simulink model "Modelo_Omnirover"  (R2026b)
settings: Solver=ode23t  StopTime=100
InitFcn:
  | %% Modelo Proyecto Omnriover - Hermes
  | clc;
  | clear;
  | 
  | % Variables de Sim
  | step_time = 1;
  | % initial_val = 10;
  | 
  | % Max Val = 7-8 rad/s
  | 
  | w1_val = 7.2; % M1 delantero izquierdo
  | w2_val = 7.2; % M2 delantero derecho
  | w3_val = 7.2; % M3 trasero izquierdo
  | w4_val = 7.2; % M4 trasero derecho
  | final_val = 0;
  | sample_time = 100;
  | 
  | % Condiciones Iniciales
  | x0 = [0; 0; 0];
  | 
  | 
  | %% PID
  | % Simulacion de Motor
  | V_nom = 12; % V
  | Vel_nom_150rpm = 100; % RPM
  | Vel_nom_140rpm = 70; % RPM
  | 
  | W_nom_150rpm = Vel_nom_150rpm * (2*pi) * (1/60);
  | W_nom_140rpm = Vel_nom_140rpm * (2*pi) * (1/60);
  | K_150 = W_nom_150rpm/V_nom;
  | K_140 = W_nom_140rpm/V_nom;
  | 
  | tao = 0.1; % entre 50 - 200 ms
  | 
  | % Ganancias PIDs
  | N = 100;
  | Kp1 = 0; % Robustez 1.5
  | Ki1 = 4.35; % 200 works
  | Kd1 = 0.005;
  | 
  | Kp2 = 0;
  | Ki2 = 3;
  | Kd2 = 0.005;
  | 
  | Kp3 = 0;
  | Ki3 = 3;
  | Kd3 = 0.005;
  | 
  | Kp4 = 0;
  | Ki4 = 3;
  | Kd4 = 0.005;
libraries: slpidlib x4
settings Model: Creator=dbarraga  LastModifiedBy=dbarraga

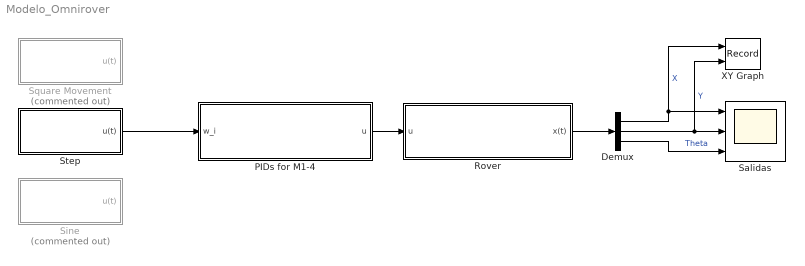
== system Modelo_Omnirover ==
  Demux : Demux  Outputs=3
  PIDs for M1-4 : Subsystem
  Rover : Subsystem
  Salidas : Scope  NumInputPorts=3
      settings: ActiveDisplayYMinimum=-3.586291147206452  ActiveDisplayYMaximum=32.276620324858079
  Sine : Subsystem  Commented=on
  Square Movement : Subsystem  Commented=on
  Step : Subsystem
  XY Graph : Record  NumPorts=2.0  FileSettingsInternal="{\"entries\":[{\"content\":{\"excelSettings\":{\"content\":{},\"type\":\"Streamout.ExcelSettings\"},\"parquetSettings\":{\"content\":{},\"type\":\"Streamout.ParquetSettings\"}},\"type\":\"Streamout.FileSettingStorage\",\"uuid\":\"\"}],\"packageUris\":[\"http:\\/\\/schema.mathworks.com\\/mf0\\/streamout_blocks\\/R2020a\"],\"version\":\"1.0\"}"  FrameSettings=[0, 0]  Layout=[1 1]  SignalsInternal="{\"entries\":[{\"content\":{\"signals\":[{\"content\":{\"blockPath\":[],\"dimensions\":[1,1],\"domain\":\"\",\"lineColor\":\"#a2142f\",\"plots\":[ 1 ],\"port\":1,\"sid\":[\"\"],\"signalID\":1,\"signalName\":\"X\"},\"type\":\"RecordBlkView.Signal\",\"uuid\":\"\"},{\"content\":{\"blockPath\":[],\"dimensions\":[1,1],\"domain\":\"\",\"lineColor\":\"#139fff\",\"plots\":[ 1 ],\"port\":2,\"sid\":[\"\"],\"signalID\":2,\"signalName\":\"Y\"},\"type\":\"RecordBlkView.Signal\",\"uuid\":\"\"}]},\"type\":\"RecordBlkView.InputSignals\",\"uuid\":\"\"}],\"packageUris\":[\"http:\\/\\/schema.mathworks.com\\/mf0\\/streamout_blocks\\/R2020a\"],\"version\":\"1.0\"}"  VisualizationBindings="{\"xyplotplugin\":{\"info\":[{\"series\":[{\"bindingParametersList\":[{\"parameter\":\"X-Axis\",\"signalID\":2,\"signalName\":\"Y\"},{\"parameter\":\"Y-Axis\",\"signalID\":1,\"signalName\":\"X\"}],\"seriesID\":0}],\"subplotID\":1}]}}"  CompatibilityTag=XY
  wires:
  Demux/2 -> XY Graph/2, Salidas/2  "Y"
  Demux/1 -> XY Graph/1, Salidas/1  "X"
  Demux/3 -> Salidas/3  "Theta"
  Rover/1(x(t)) -> Demux/1
  PIDs for M1-4/1(u) -> Rover/1(u)
  Step/1(u(t)) -> PIDs for M1-4/1(w_i)

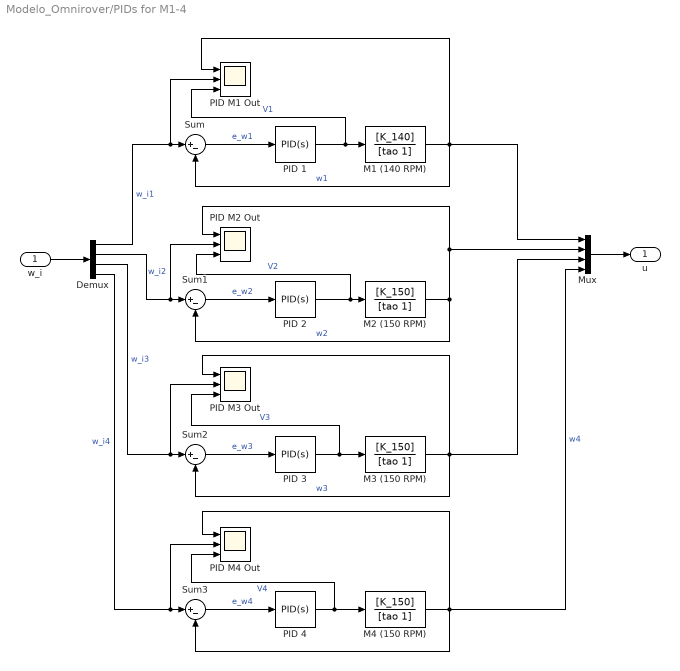
== system Modelo_Omnirover/PIDs for M1-4 ==
  w_i : Inport
  Demux : Demux
  M1 (140 RPM) : TransferFcn  Numerator=[K_140]  Denominator=[tao 1]
  M2 (150 RPM) : TransferFcn  Numerator=[K_150]  Denominator=[tao 1]
  M3 (150 RPM) : TransferFcn  Numerator=[K_150]  Denominator=[tao 1]
  M4 (150 RPM) : TransferFcn  Numerator=[K_150]  Denominator=[tao 1]
  Mux : Mux
  PID 1 : slpidlib/PID Controller  Controller=PID  Form=Parallel  TimeDomain=Continuous-time  UseExternalTs=off  SampleTime=-1  IntegratorMethod=Forward Euler  FilterMethod=Forward Euler  ControllerParametersSource=internal  P=Kp1  I=Ki1  UseKiTs=off  D=Kd1  UseExternalDerivativeSource=off  N=N  UseFilter=on  TunerSelectOption=Transfer Function Based (PID Tuner App)  InitialConditionSource=internal  InitialConditionForIntegrator=0  InitialConditionForFilter=0  DifferentiatorICPrevScaledInput=0  ExternalReset=none  TrackingMode=off  Kt=1  LimitOutput=off  SatLimitsSource=internal  UpperSaturationLimit=inf  LowerSaturationLimit=-inf  LinearizeAsGain=on  AntiWindupMode=none  Kb=1  LimitIntegrator=off  UpperIntegratorSaturationLimit=inf  LowerIntegratorSaturationLimit=-inf  POutMin=[]  POutMax=[]  IOutMin=[]  IOutMax=[]  DOutMin=[]  DOutMax=[]  NOutMin=[]  NOutMax=[]  SumOutMin=[]  SumOutMax=[]  SaturationOutMin=[]  SaturationOutMax=[]  PParamMin=[]  PParamMax=[]  IParamMin=[]  IParamMax=[]  DParamMin=[]  DParamMax=[]  NParamMin=[]  NParamMax=[]  KbParamMin=[]  KbParamMax=[]  KtParamMin=[]  KtParamMax=[]  KbOutMin=[]  KbOutMax=[]  KtOutMin=[]  KtOutMax=[]  IntegratorOutMin=[]  IntegratorOutMax=[]  FilterOutMin=[]  FilterOutMax=[]  SumI1OutMin=[]  SumI1OutMax=[]  SumI2OutMin=[]  SumI2OutMax=[]  SumI3OutMin=[]  SumI3OutMax=[]  SumI4OutMin=[]  SumI4OutMax=[]  SumDOutMin=[]  SumDOutMax=[]  DifferentiatorOutMin=[]  DifferentiatorOutMax=[]  FilterDiffOutCoefMin=[]  FilterDiffOutCoefMax=[]  ReciprocalOutMin=[]  ReciprocalOutMax=[]  SumDenOutMin=[]  SumDenOutMax=[]  SumNumOutMin=[]  SumNumOutMax=[]  DivideOutMin=[]  DivideOutMax=[]  UdiffTsProdOutMin=[]  UdiffTsProdOutMax=[]  NTsProdOutMin=[]  NTsProdOutMax=[]  UintegralTsProdOutMin=[]  UintegralTsProdOutMax=[]  UngainTsProdOutMin=[]  UngainTsProdOutMax=[]  ClampingZeroOutDataTypeStr=Inherit: Inherit via back propagation  ClampingZeroOutMin=[]  ClampingZeroOutMax=[]  FilterDenConstantOutDataTypeStr=Inherit: Inherit via back propagation  FilterDenConstantOutMin=[]  FilterDenConstantOutMax=[]  PCopyOutDataTypeStr=Inherit: Inherit via back propagation  PCopyOutMin=[]  PCopyOutMax=[]  NCopyOutDataTypeStr=Inherit: Inherit via back propagation  NCopyOutMin=[]  NCopyOutMax=[]  IntegratorContinuousStateAttributes=''  IntegratorStateMustResolveToSignalObject=off  IntegratorRTWStateStorageClass=Auto  FilterContinuousStateAttributes=''  FilterStateMustResolveToSignalObject=off  FilterRTWStateStorageClass=Auto  ParallelPVariant=InternalParameters  IdealPVariant=Disabled  IVariant=InternalParameters  DVariant=InternalParameters  IntegratorVariant=Continuous  SatVariant=Disabled  AWVariant=Passthrough  PCopyVariant=Disabled  TRVariant=Disabled  FdbkBlocksVariant=Forward  IdealPFdbkVariant=Disabled  SatFdbkVariant=Disabled  DerivativeFilterVariant=ContFilter  NVariant=InternalParameters  NCopyVariant=Disabled  FilterICVariant=InternalICsFilter  IntegratorICVariant=InternalICs  ExternalResetVariant=Disabled  TRSumVariant=Passthrough  SumFdbkVariant=Disabled  SumVariant=Sum_PID  TsampFilterVariant=InternalTs  TsampNgainVariant=Passthrough  TsampIntegralVariant=Disabled_SignalSpec  ExternalSaturationOutDataTypeStr=Inherit: Same as second input  DerivativeSourceVariant=ErrorSignal  PreIntVariant=InternalPreInt
  PID 2 : slpidlib/PID Controller  Controller=PID  Form=Parallel  TimeDomain=Continuous-time  UseExternalTs=off  SampleTime=-1  IntegratorMethod=Forward Euler  FilterMethod=Forward Euler  ControllerParametersSource=internal  P=Kp2  I=Ki2  UseKiTs=off  D=Kd2  UseExternalDerivativeSource=off  N=N  UseFilter=on  TunerSelectOption=Transfer Function Based (PID Tuner App)  InitialConditionSource=internal  InitialConditionForIntegrator=0  InitialConditionForFilter=0  DifferentiatorICPrevScaledInput=0  ExternalReset=none  TrackingMode=off  Kt=1  LimitOutput=off  SatLimitsSource=internal  UpperSaturationLimit=inf  LowerSaturationLimit=-inf  LinearizeAsGain=on  AntiWindupMode=none  Kb=1  LimitIntegrator=off  UpperIntegratorSaturationLimit=inf  LowerIntegratorSaturationLimit=-inf  POutMin=[]  POutMax=[]  IOutMin=[]  IOutMax=[]  DOutMin=[]  DOutMax=[]  NOutMin=[]  NOutMax=[]  SumOutMin=[]  SumOutMax=[]  SaturationOutMin=[]  SaturationOutMax=[]  PParamMin=[]  PParamMax=[]  IParamMin=[]  IParamMax=[]  DParamMin=[]  DParamMax=[]  NParamMin=[]  NParamMax=[]  KbParamMin=[]  KbParamMax=[]  KtParamMin=[]  KtParamMax=[]  KbOutMin=[]  KbOutMax=[]  KtOutMin=[]  KtOutMax=[]  IntegratorOutMin=[]  IntegratorOutMax=[]  FilterOutMin=[]  FilterOutMax=[]  SumI1OutMin=[]  SumI1OutMax=[]  SumI2OutMin=[]  SumI2OutMax=[]  SumI3OutMin=[]  SumI3OutMax=[]  SumI4OutMin=[]  SumI4OutMax=[]  SumDOutMin=[]  SumDOutMax=[]  DifferentiatorOutMin=[]  DifferentiatorOutMax=[]  FilterDiffOutCoefMin=[]  FilterDiffOutCoefMax=[]  ReciprocalOutMin=[]  ReciprocalOutMax=[]  SumDenOutMin=[]  SumDenOutMax=[]  SumNumOutMin=[]  SumNumOutMax=[]  DivideOutMin=[]  DivideOutMax=[]  UdiffTsProdOutMin=[]  UdiffTsProdOutMax=[]  NTsProdOutMin=[]  NTsProdOutMax=[]  UintegralTsProdOutMin=[]  UintegralTsProdOutMax=[]  UngainTsProdOutMin=[]  UngainTsProdOutMax=[]  ClampingZeroOutDataTypeStr=Inherit: Inherit via back propagation  ClampingZeroOutMin=[]  ClampingZeroOutMax=[]  FilterDenConstantOutDataTypeStr=Inherit: Inherit via back propagation  FilterDenConstantOutMin=[]  FilterDenConstantOutMax=[]  PCopyOutDataTypeStr=Inherit: Inherit via back propagation  PCopyOutMin=[]  PCopyOutMax=[]  NCopyOutDataTypeStr=Inherit: Inherit via back propagation  NCopyOutMin=[]  NCopyOutMax=[]  IntegratorContinuousStateAttributes=''  IntegratorStateMustResolveToSignalObject=off  IntegratorRTWStateStorageClass=Auto  FilterContinuousStateAttributes=''  FilterStateMustResolveToSignalObject=off  FilterRTWStateStorageClass=Auto  ParallelPVariant=InternalParameters  IdealPVariant=Disabled  IVariant=InternalParameters  DVariant=InternalParameters  IntegratorVariant=Continuous  SatVariant=Disabled  AWVariant=Passthrough  PCopyVariant=Disabled  TRVariant=Disabled  FdbkBlocksVariant=Forward  IdealPFdbkVariant=Disabled  SatFdbkVariant=Disabled  DerivativeFilterVariant=ContFilter  NVariant=InternalParameters  NCopyVariant=Disabled  FilterICVariant=InternalICsFilter  IntegratorICVariant=InternalICs  ExternalResetVariant=Disabled  TRSumVariant=Passthrough  SumFdbkVariant=Disabled  SumVariant=Sum_PID  TsampFilterVariant=InternalTs  TsampNgainVariant=Passthrough  TsampIntegralVariant=Disabled_SignalSpec  ExternalSaturationOutDataTypeStr=Inherit: Same as second input  DerivativeSourceVariant=ErrorSignal  PreIntVariant=InternalPreInt
  PID 3 : slpidlib/PID Controller  Controller=PID  Form=Parallel  TimeDomain=Continuous-time  UseExternalTs=off  SampleTime=-1  IntegratorMethod=Forward Euler  FilterMethod=Forward Euler  ControllerParametersSource=internal  P=Kp3  I=Ki3  UseKiTs=off  D=Kd3  UseExternalDerivativeSource=off  N=N  UseFilter=on  TunerSelectOption=Transfer Function Based (PID Tuner App)  InitialConditionSource=internal  InitialConditionForIntegrator=0  InitialConditionForFilter=0  DifferentiatorICPrevScaledInput=0  ExternalReset=none  TrackingMode=off  Kt=1  LimitOutput=off  SatLimitsSource=internal  UpperSaturationLimit=inf  LowerSaturationLimit=-inf  LinearizeAsGain=on  AntiWindupMode=none  Kb=1  LimitIntegrator=off  UpperIntegratorSaturationLimit=inf  LowerIntegratorSaturationLimit=-inf  POutMin=[]  POutMax=[]  IOutMin=[]  IOutMax=[]  DOutMin=[]  DOutMax=[]  NOutMin=[]  NOutMax=[]  SumOutMin=[]  SumOutMax=[]  SaturationOutMin=[]  SaturationOutMax=[]  PParamMin=[]  PParamMax=[]  IParamMin=[]  IParamMax=[]  DParamMin=[]  DParamMax=[]  NParamMin=[]  NParamMax=[]  KbParamMin=[]  KbParamMax=[]  KtParamMin=[]  KtParamMax=[]  KbOutMin=[]  KbOutMax=[]  KtOutMin=[]  KtOutMax=[]  IntegratorOutMin=[]  IntegratorOutMax=[]  FilterOutMin=[]  FilterOutMax=[]  SumI1OutMin=[]  SumI1OutMax=[]  SumI2OutMin=[]  SumI2OutMax=[]  SumI3OutMin=[]  SumI3OutMax=[]  SumI4OutMin=[]  SumI4OutMax=[]  SumDOutMin=[]  SumDOutMax=[]  DifferentiatorOutMin=[]  DifferentiatorOutMax=[]  FilterDiffOutCoefMin=[]  FilterDiffOutCoefMax=[]  ReciprocalOutMin=[]  ReciprocalOutMax=[]  SumDenOutMin=[]  SumDenOutMax=[]  SumNumOutMin=[]  SumNumOutMax=[]  DivideOutMin=[]  DivideOutMax=[]  UdiffTsProdOutMin=[]  UdiffTsProdOutMax=[]  NTsProdOutMin=[]  NTsProdOutMax=[]  UintegralTsProdOutMin=[]  UintegralTsProdOutMax=[]  UngainTsProdOutMin=[]  UngainTsProdOutMax=[]  ClampingZeroOutDataTypeStr=Inherit: Inherit via back propagation  ClampingZeroOutMin=[]  ClampingZeroOutMax=[]  FilterDenConstantOutDataTypeStr=Inherit: Inherit via back propagation  FilterDenConstantOutMin=[]  FilterDenConstantOutMax=[]  PCopyOutDataTypeStr=Inherit: Inherit via back propagation  PCopyOutMin=[]  PCopyOutMax=[]  NCopyOutDataTypeStr=Inherit: Inherit via back propagation  NCopyOutMin=[]  NCopyOutMax=[]  IntegratorContinuousStateAttributes=''  IntegratorStateMustResolveToSignalObject=off  IntegratorRTWStateStorageClass=Auto  FilterContinuousStateAttributes=''  FilterStateMustResolveToSignalObject=off  FilterRTWStateStorageClass=Auto  ParallelPVariant=InternalParameters  IdealPVariant=Disabled  IVariant=InternalParameters  DVariant=InternalParameters  IntegratorVariant=Continuous  SatVariant=Disabled  AWVariant=Passthrough  PCopyVariant=Disabled  TRVariant=Disabled  FdbkBlocksVariant=Forward  IdealPFdbkVariant=Disabled  SatFdbkVariant=Disabled  DerivativeFilterVariant=ContFilter  NVariant=InternalParameters  NCopyVariant=Disabled  FilterICVariant=InternalICsFilter  IntegratorICVariant=InternalICs  ExternalResetVariant=Disabled  TRSumVariant=Passthrough  SumFdbkVariant=Disabled  SumVariant=Sum_PID  TsampFilterVariant=InternalTs  TsampNgainVariant=Passthrough  TsampIntegralVariant=Disabled_SignalSpec  ExternalSaturationOutDataTypeStr=Inherit: Same as second input  DerivativeSourceVariant=ErrorSignal  PreIntVariant=InternalPreInt
  PID 4 : slpidlib/PID Controller  Controller=PID  Form=Parallel  TimeDomain=Continuous-time  UseExternalTs=off  SampleTime=-1  IntegratorMethod=Forward Euler  FilterMethod=Forward Euler  ControllerParametersSource=internal  P=Kp4  I=Ki4  UseKiTs=off  D=Kd4  UseExternalDerivativeSource=off  N=N  UseFilter=on  TunerSelectOption=Transfer Function Based (PID Tuner App)  InitialConditionSource=internal  InitialConditionForIntegrator=0  InitialConditionForFilter=0  DifferentiatorICPrevScaledInput=0  ExternalReset=none  TrackingMode=off  Kt=1  LimitOutput=off  SatLimitsSource=internal  UpperSaturationLimit=inf  LowerSaturationLimit=-inf  LinearizeAsGain=on  AntiWindupMode=none  Kb=1  LimitIntegrator=off  UpperIntegratorSaturationLimit=inf  LowerIntegratorSaturationLimit=-inf  POutMin=[]  POutMax=[]  IOutMin=[]  IOutMax=[]  DOutMin=[]  DOutMax=[]  NOutMin=[]  NOutMax=[]  SumOutMin=[]  SumOutMax=[]  SaturationOutMin=[]  SaturationOutMax=[]  PParamMin=[]  PParamMax=[]  IParamMin=[]  IParamMax=[]  DParamMin=[]  DParamMax=[]  NParamMin=[]  NParamMax=[]  KbParamMin=[]  KbParamMax=[]  KtParamMin=[]  KtParamMax=[]  KbOutMin=[]  KbOutMax=[]  KtOutMin=[]  KtOutMax=[]  IntegratorOutMin=[]  IntegratorOutMax=[]  FilterOutMin=[]  FilterOutMax=[]  SumI1OutMin=[]  SumI1OutMax=[]  SumI2OutMin=[]  SumI2OutMax=[]  SumI3OutMin=[]  SumI3OutMax=[]  SumI4OutMin=[]  SumI4OutMax=[]  SumDOutMin=[]  SumDOutMax=[]  DifferentiatorOutMin=[]  DifferentiatorOutMax=[]  FilterDiffOutCoefMin=[]  FilterDiffOutCoefMax=[]  ReciprocalOutMin=[]  ReciprocalOutMax=[]  SumDenOutMin=[]  SumDenOutMax=[]  SumNumOutMin=[]  SumNumOutMax=[]  DivideOutMin=[]  DivideOutMax=[]  UdiffTsProdOutMin=[]  UdiffTsProdOutMax=[]  NTsProdOutMin=[]  NTsProdOutMax=[]  UintegralTsProdOutMin=[]  UintegralTsProdOutMax=[]  UngainTsProdOutMin=[]  UngainTsProdOutMax=[]  ClampingZeroOutDataTypeStr=Inherit: Inherit via back propagation  ClampingZeroOutMin=[]  ClampingZeroOutMax=[]  FilterDenConstantOutDataTypeStr=Inherit: Inherit via back propagation  FilterDenConstantOutMin=[]  FilterDenConstantOutMax=[]  PCopyOutDataTypeStr=Inherit: Inherit via back propagation  PCopyOutMin=[]  PCopyOutMax=[]  NCopyOutDataTypeStr=Inherit: Inherit via back propagation  NCopyOutMin=[]  NCopyOutMax=[]  IntegratorContinuousStateAttributes=''  IntegratorStateMustResolveToSignalObject=off  IntegratorRTWStateStorageClass=Auto  FilterContinuousStateAttributes=''  FilterStateMustResolveToSignalObject=off  FilterRTWStateStorageClass=Auto  ParallelPVariant=InternalParameters  IdealPVariant=Disabled  IVariant=InternalParameters  DVariant=InternalParameters  IntegratorVariant=Continuous  SatVariant=Disabled  AWVariant=Passthrough  PCopyVariant=Disabled  TRVariant=Disabled  FdbkBlocksVariant=Forward  IdealPFdbkVariant=Disabled  SatFdbkVariant=Disabled  DerivativeFilterVariant=ContFilter  NVariant=InternalParameters  NCopyVariant=Disabled  FilterICVariant=InternalICsFilter  IntegratorICVariant=InternalICs  ExternalResetVariant=Disabled  TRSumVariant=Passthrough  SumFdbkVariant=Disabled  SumVariant=Sum_PID  TsampFilterVariant=InternalTs  TsampNgainVariant=Passthrough  TsampIntegralVariant=Disabled_SignalSpec  ExternalSaturationOutDataTypeStr=Inherit: Same as second input  DerivativeSourceVariant=ErrorSignal  PreIntVariant=InternalPreInt
  PID M1 Out : Scope  NumInputPorts=3
      settings: ActiveDisplayYMinimum=-1.4313542038944647  ActiveDisplayYMaximum=12.882187835050184
  PID M2 Out : Scope  NumInputPorts=3
      settings: ActiveDisplayYMinimum=-1.0027273876397875  ActiveDisplayYMaximum=9.0245464887580891  DataLoggingVariableName=ScopeData2
  PID M3 Out : Scope  NumInputPorts=3
      settings: ActiveDisplayYMinimum=-1  ActiveDisplayYMaximum=1  DataLoggingVariableName=ScopeData3
  PID M4 Out : Scope  NumInputPorts=3
      settings: ActiveDisplayYMinimum=-1.4324857395617314  ActiveDisplayYMaximum=12.892371656055584  DataLoggingVariableName=ScopeData4
  Sum{,1..3} (4 alike) : Sum  Inputs=|+-
  u : Outport
  wires:
  Sum/1 -> PID 1/1  "e_w1"
  Demux/1 -> PID M1 Out/2, Sum/1  "w_i1"
  M1 (140 RPM)/1 -> PID M1 Out/1, Mux/1, Sum/2  "w1"
  Sum1/1 -> PID 2/1  "e_w2"
  M2 (150 RPM)/1 -> Sum1/2, PID M2 Out/1, Mux/2  "w2"
  PID 2/1 -> PID M2 Out/3, M2 (150 RPM)/1  "V2"
  Demux/2 -> PID M2 Out/2, Sum1/1  "w_i2"
  Sum3/1 -> PID 4/1  "e_w4"
  M4 (150 RPM)/1 -> PID M4 Out/1, Mux/4, Sum3/2  "w4"
  Sum2/1 -> PID 3/1  "e_w3"
  PID 4/1 -> PID M4 Out/3, M4 (150 RPM)/1  "V4"
  M3 (150 RPM)/1 -> PID M3 Out/1, Mux/3, Sum2/2  "w3"
  PID 3/1 -> PID M3 Out/3, M3 (150 RPM)/1  "V3"
  Demux/3 -> PID M3 Out/2, Sum2/1  "w_i3"
  Demux/4 -> PID M4 Out/2, Sum3/1  "w_i4"
  w_i/1 -> Demux/1
  Mux/1 -> u/1
  PID 1/1 -> M1 (140 RPM)/1, PID M1 Out/3  "V1"

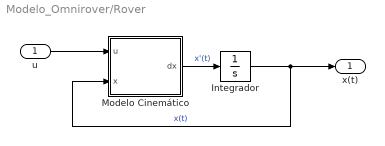
== system Modelo_Omnirover/Rover ==
  u : Inport
  "Integrador " : Integrator  InitialCondition=x0
  Modelo Cinemático : MATLAB Function  TreatAsAtomicUnit=on
  x(t) : Outport
  wires:
  Modelo Cinemático/1(dx) -> "Integrador "/1  "x'(t)"
  "Integrador "/1 -> x(t)/1, Modelo Cinemático/2(x)  "x(t)"
  u/1 -> Modelo Cinemático/1(u)

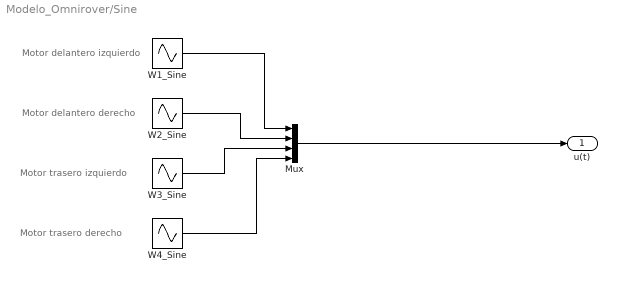
== system Modelo_Omnirover/Sine ==
  note: Motor delantero izquierdo
  note: Motor delantero derecho
  note: Motor trasero izquierdo
  note: Motor trasero derecho
  Mux : Mux
  W1_Sine : Sin  SampleTime=0
  W2_Sine : Sin  SampleTime=0
  W3_Sine : Sin  SampleTime=0
  W4_Sine : Sin  SampleTime=0
  u(t) : Outport
  wires:
  Mux/1 -> u(t)/1
  W2_Sine/1 -> Mux/2
  W1_Sine/1 -> Mux/1
  W3_Sine/1 -> Mux/3
  W4_Sine/1 -> Mux/4

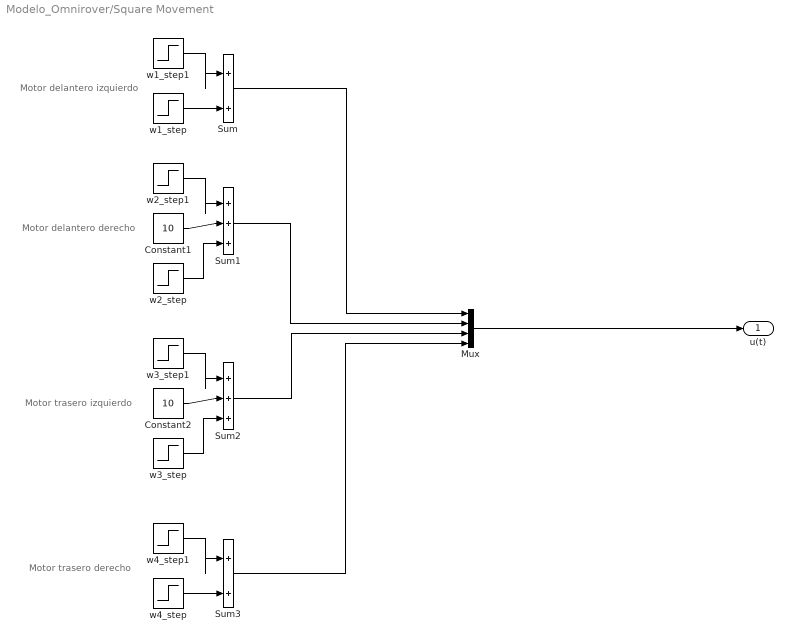
== system Modelo_Omnirover/Square Movement ==
  note: Motor trasero izquierdo
  note: Motor delantero izquierdo
  note: Motor delantero derecho
  note: Motor trasero derecho
  Constant1 : Constant  Value=10
  Constant2 : Constant  Value=10
  Mux : Mux
  Sum : Sum  Inputs=|++
  Sum1 : Sum  Inputs=|+++
  Sum2 : Sum  Inputs=|+++
  Sum3 : Sum  Inputs=|++
  w1_step : Step  Time=step_time  FinalValue=-10  SampleTime=50
  w1_step1 : Step  Time=step_time  InitialValue=10  FinalValue=0  SampleTime=50
  w2_step : Step  Time=step_time  FinalValue=20  SampleTime=75
  w2_step1 : Step  Time=step_time  FinalValue=-20  SampleTime=25
  w3_step : Step  Time=step_time  FinalValue=20  SampleTime=75
  w3_step1 : Step  Time=step_time  FinalValue=-20  SampleTime=25
  w4_step : Step  Time=step_time  FinalValue=-10  SampleTime=50
  w4_step1 : Step  Time=step_time  InitialValue=10  FinalValue=0  SampleTime=50
  u(t) : Outport
  wires:
  Mux/1 -> u(t)/1
  w1_step1/1 -> Sum/1
  w1_step/1 -> Sum/2
  Constant1/1 -> Sum1/2
  w2_step1/1 -> Sum1/1
  w2_step/1 -> Sum1/3
  Constant2/1 -> Sum2/2
  w3_step1/1 -> Sum2/1
  w3_step/1 -> Sum2/3
  w4_step/1 -> Sum3/2
  w4_step1/1 -> Sum3/1
  Sum/1 -> Mux/1
  Sum1/1 -> Mux/2
  Sum2/1 -> Mux/3
  Sum3/1 -> Mux/4

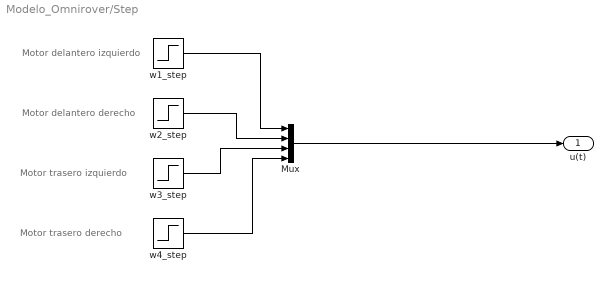
== system Modelo_Omnirover/Step ==
  note: Motor trasero izquierdo
  note: Motor delantero izquierdo
  note: Motor delantero derecho
  note: Motor trasero derecho
  Mux : Mux
  w1_step : Step  Time=step_time  InitialValue=w1_val  FinalValue=final_val  SampleTime=sample_time
  w2_step : Step  Time=step_time  InitialValue=w2_val  FinalValue=final_val  SampleTime=sample_time
  w3_step : Step  Time=step_time  InitialValue=w3_val  FinalValue=final_val  SampleTime=sample_time
  w4_step : Step  Time=step_time  InitialValue=w4_val  FinalValue=final_val  SampleTime=sample_time
  u(t) : Outport
  wires:
  Mux/1 -> u(t)/1
  w2_step/1 -> Mux/2
  w1_step/1 -> Mux/1
  w3_step/1 -> Mux/3
  w4_step/1 -> Mux/4

== matlab function Modelo_Omnirover/Rover/Modelo Cinemático ==
  data: u input; dx output; x input
function dx = m_c(u, x)
% Definición de parámetros físicos del SAOAH
Rw = 0.04;    % Radio de la rueda Mecanum en m (80mm diámetro)
L  = 0.08;    % Distancia del centro de masa al eje Y en m
l  = 0.105;   % Distancia del centro de masa al eje X en m (incluye acoples)

% Extracción de la orientación actual
% El vector x contiene [posición_x, posición_y, angulo_theta]
theta = x(3);

% Matriz de acoplamiento de las 4 ruedas (J)
J = (Rw/4) * [  1,        1,        1,        1;
    -1,        1,        1,       -1;
    -1/(L+l),  1/(L+l), -1/(L+l),  1/(L+l)];

% Matriz de rotación global (R)
R = [ cos(theta), -sin(theta), 0;
    sin(theta),  cos(theta), 0;
    0,           0,          1 ];

% Cálculo de la EDO no lineal (dx = R * J * u)
dx = R * J * u;
